simulink model "PINN_Fuzzy_HEV"  (R2024b)
settings: Solver=VariableStepAuto  StartTime=0.0  StopTime=0.1  RelTol=1e-3
settings Model: Creator=Admin  LastModifiedBy=Admin

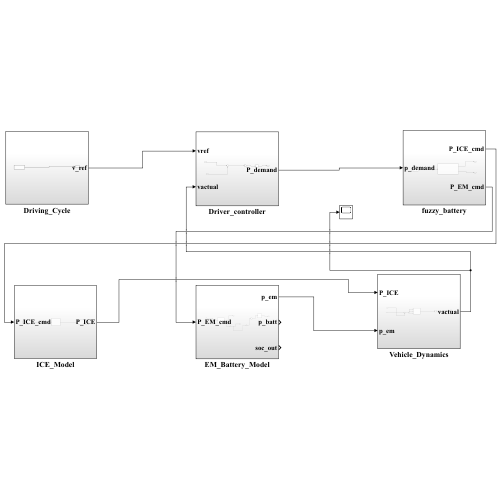
[thumbnail: Simulink's stored preview of the top-level diagram]
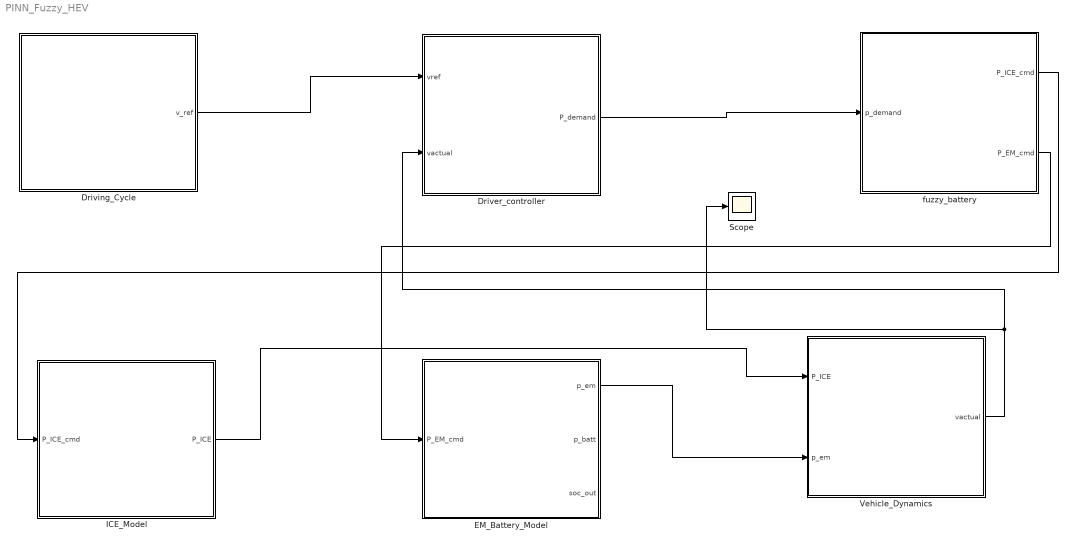
== system PINN_Fuzzy_HEV ==
  Driver_controller : Subsystem
  Driving_Cycle : Subsystem
  EM_Battery_Model : Subsystem
  ICE_Model : Subsystem
  Scope : Scope
  Vehicle_Dynamics : Subsystem
  fuzzy_battery : Subsystem
  wires:
  Driver_controller/1(P_demand) -> fuzzy_battery/1(p_demand)
  fuzzy_battery/1(P_ICE_cmd) -> ICE_Model/1(P_ICE_cmd)
  fuzzy_battery/2(P_EM_cmd) -> EM_Battery_Model/1(P_EM_cmd)
  Driving_Cycle/1(v_ref) -> Driver_controller/1(vref)
  ICE_Model/1(P_ICE) -> Vehicle_Dynamics/1(P_ICE)
  Vehicle_Dynamics/1(vactual) -> Scope/1, Driver_controller/2(vactual)
  EM_Battery_Model/1(p_em) -> Vehicle_Dynamics/2(p_em)

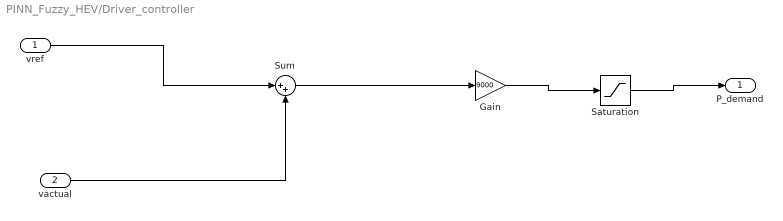
== system PINN_Fuzzy_HEV/Driver_controller ==
  vref : Inport
  vactual : Inport  Port=2
  Gain : Gain  Gain=9000
  Saturation : Saturate  UpperLimit=75000  LowerLimit=0
  Sum : Sum  Inputs=|++
  P_demand : Outport
  wires:
  vref/1 -> Sum/1
  vactual/1 -> Sum/2
  Sum/1 -> Gain/1
  Gain/1 -> Saturation/1
  Saturation/1 -> P_demand/1

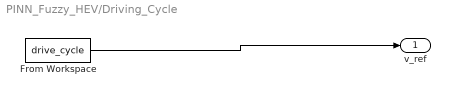
== system PINN_Fuzzy_HEV/Driving_Cycle ==
  From Workspace : FromWorkspace  VariableName=drive_cycle  SampleTime=1
  v_ref : Outport
  wires:
  From Workspace/1 -> v_ref/1

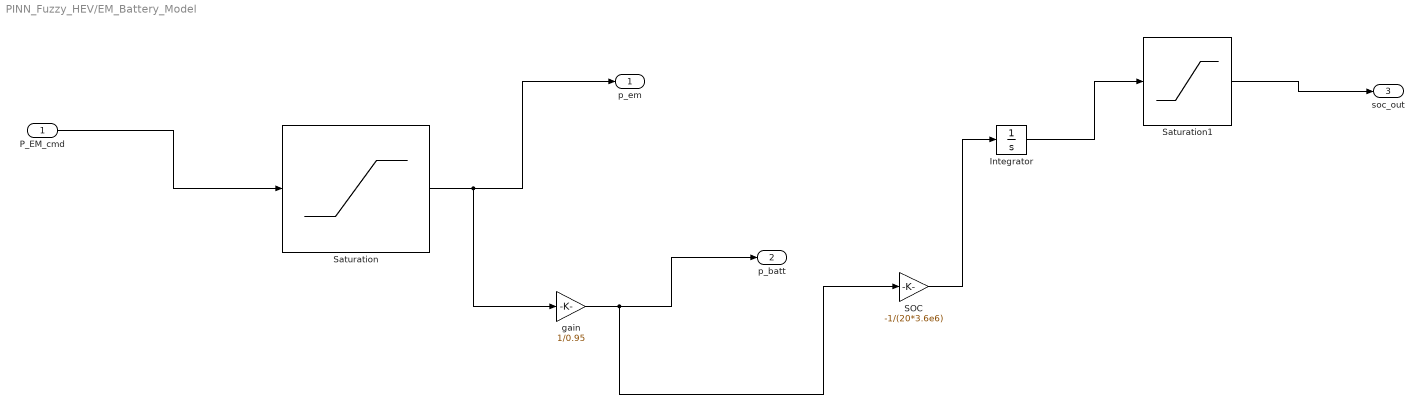
== system PINN_Fuzzy_HEV/EM_Battery_Model ==
  P_EM_cmd : Inport
  Integrator : Integrator  InitialCondition=0.6
  SOC : Gain  Gain=-1/(20*3.6e6)
  Saturation : Saturate  UpperLimit=50000  LowerLimit=0
  Saturation1 : Saturate  UpperLimit=1  LowerLimit=0
  gain : Gain  Gain=1/0.95
  p_em : Outport
  p_batt : Outport  Port=2
  soc_out : Outport  Port=3
  wires:
  P_EM_cmd/1 -> Saturation/1
  Saturation/1 -> gain/1, p_em/1
  gain/1 -> SOC/1, p_batt/1
  SOC/1 -> Integrator/1
  Integrator/1 -> Saturation1/1
  Saturation1/1 -> soc_out/1

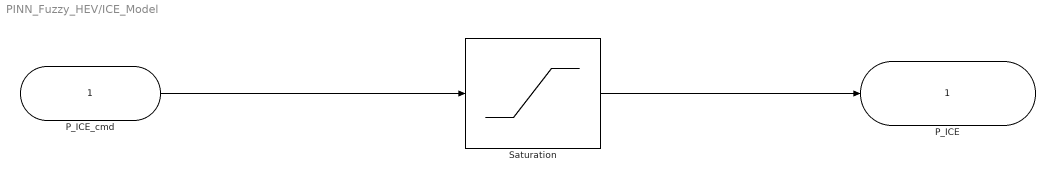
== system PINN_Fuzzy_HEV/ICE_Model ==
  P_ICE_cmd : Inport
  Saturation : Saturate  UpperLimit=75000  LowerLimit=0
  P_ICE : Outport
  wires:
  P_ICE_cmd/1 -> Saturation/1
  Saturation/1 -> P_ICE/1

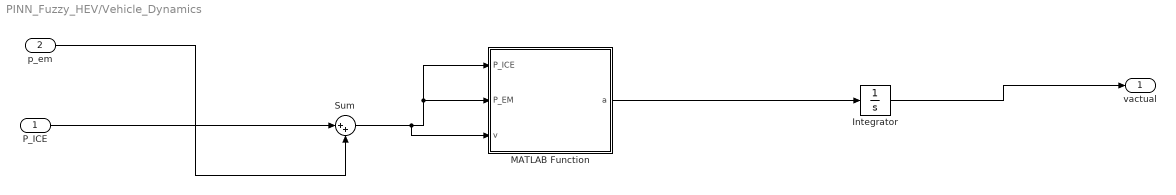
== system PINN_Fuzzy_HEV/Vehicle_Dynamics ==
  P_ICE : Inport
  p_em : Inport  Port=2
  Integrator : Integrator
  MATLAB Function : MATLAB Function  TreatAsAtomicUnit=on
  Sum : Sum  Inputs=|++
  vactual : Outport
  wires:
  P_ICE/1 -> Sum/1
  MATLAB Function/1(a) -> Integrator/1
  Integrator/1 -> vactual/1
  p_em/1 -> Sum/2
  Sum/1 -> MATLAB Function/3(v), MATLAB Function/1(P_ICE), MATLAB Function/2(P_EM)

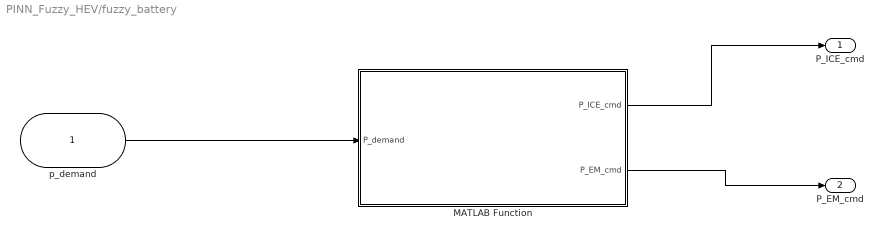
== system PINN_Fuzzy_HEV/fuzzy_battery ==
  p_demand : Inport
  MATLAB Function : MATLAB Function  TreatAsAtomicUnit=on
  P_ICE_cmd : Outport
  P_EM_cmd : Outport  Port=2
  wires:
  p_demand/1 -> MATLAB Function/1(P_demand)
  MATLAB Function/1(P_ICE_cmd) -> P_ICE_cmd/1
  MATLAB Function/2(P_EM_cmd) -> P_EM_cmd/1

== matlab function PINN_Fuzzy_HEV/fuzzy_battery/MATLAB Function ==
  data: P_demand input; P_ICE_cmd output; P_EM_cmd output
function [P_ICE_cmd, P_EM_cmd] = fcn(P_demand)

% Non-negative power demand
P_demand = max(P_demand, 0);

% Temporary rule-based power splitting
P_ICE_cmd = 0.6 * P_demand;
P_EM_cmd  = 0.4 * P_demand;

% ICE maximum power limit
P_ICE_cmd = min(P_ICE_cmd, 75000);

end

== matlab function PINN_Fuzzy_HEV/Vehicle_Dynamics/MATLAB Function ==
  data: P_ICE input; a output; P_EM input; v input
function a = vehicle_accel(P_ICE, P_EM, v)

% Illustrative vehicle parameters
m = 1500;       % Vehicle mass (kg)
eta = 0.90;     % Drivetrain efficiency
Crr = 0.012;    % Rolling resistance coefficient
g = 9.81;       % Gravity (m/s^2)
rho = 1.225;    % Air density (kg/m^3)
Cd = 0.30;      % Drag coefficient
A = 2.2;        % Frontal area (m^2)

% Total positive traction power
P = max(P_ICE, 0) + max(P_EM, 0);

% Prevent division by zero at low speed
v_safe = max(v, 1);

% Traction force
F_traction = eta * P / v_safe;

% Road resistance
F_roll = m * g * Crr;
F_drag = 0.5 * rho * Cd * A * v^2;

% Longitudinal acceleration
a = (F_traction - F_roll - F_drag) / m;

end
